simulink model "comparisonsPID"  (R2022b)
settings: Solver=ode45  StartTime=0.0  StopTime=80000  FixedStep=1e-6  RelTol=1e-10  AbsTol=1e-10
settings Model: Creator=svens  LastModifiedBy=saraa
settings SolverCC: ZeroCrossAlgorithm=Adaptive
settings DebuggingCC: IgnoredZcDiagnostic=none

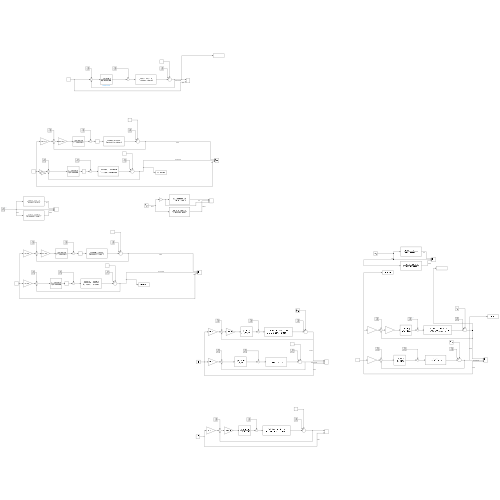
[thumbnail: Simulink's stored preview of the top-level diagram]
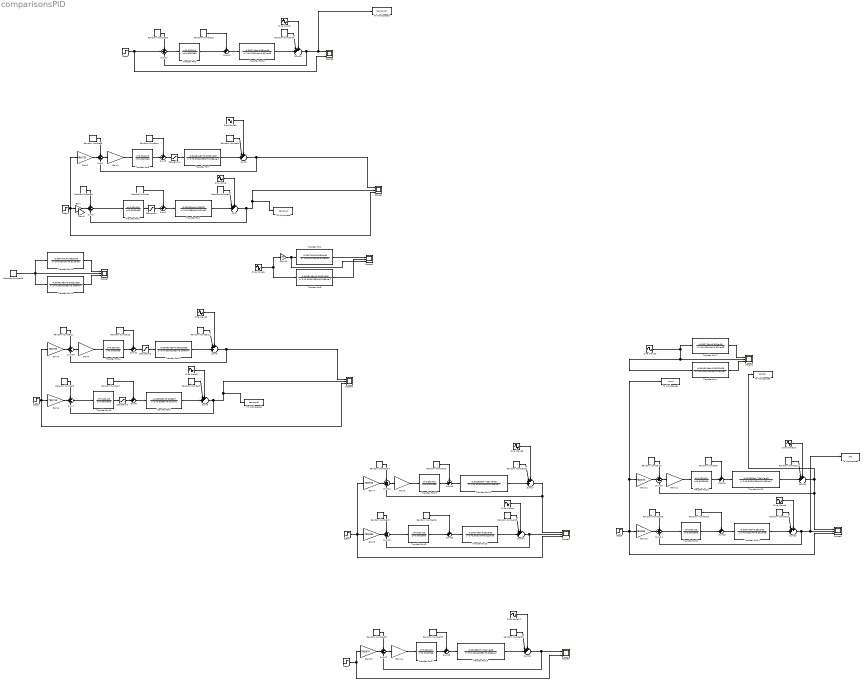
== system comparisonsPID ==
  Gain : Gain  Gain=1.05
  Gain{1,3..4,11,14} (5 alike) : Gain  Gain=0.0032072
  Gain10 : Gain  Gain=780
  Gain12 : Gain  Gain=780/675
  Gain13 : Gain  Gain=780/365
  Gain15 : Gain  Gain=780/675
  Gain2 : Gain  Gain=780/735
  Gain5 : Gain  Gain=780/735
  Gain6 : Gain  Gain=780/745
  Gain7 : Gain  Gain=780/675
  Gain8 : Gain  Gain=780/365
  Gain9 : Gain  Gain=1.05
  Random Number{,1,3..5,7..8,10..11,13..14,16..17,19..20,22..23,25..26,28..29} (21 alike) : RandomNumber  Variance=20  SampleTime=0.1
  Random Number{2,6,9,12,15,18,21,24,27,30} (10 alike) : RandomNumber  Variance=20  SampleTime=7800
  Saturation : Saturate  UpperLimit=100000  LowerLimit=50
  Saturation1 : Saturate  UpperLimit=2  LowerLimit=0  LinearizeAsGain=off
  Saturation2 : Saturate  UpperLimit=100000  LowerLimit=-10000
  Saturation3 : Saturate  UpperLimit=2  LowerLimit=0  LinearizeAsGain=off
  Scope{1..5,7..8} (7 alike) : Scope  NumInputPorts=3
  Scope6 : Scope  NumInputPorts=2
  Scope9 : Scope  NumInputPorts=2
  Sine Wave{,1..5,7..8,10,12} (10 alike) : Sin  Amplitude=6  Bias=25  Frequency=7.2e-5  SampleTime=0
  Sine Wave6 : Sin  SampleTime=0
  Sine Wave9 : Sin  SampleTime=0
  Step{1..6} (6 alike) : Step  After=780  SampleTime=0
  Sum{,3,6,9,14,17,20,23,26,32} (10 alike) : Sum  Inputs=+++||
  Sum{1,4,7,10,12,15,18,21,24,27} (10 alike) : Sum  Inputs=++-
  Sum{2,5,8,11,13,16,19,22,25,28} (10 alike) : Sum  Inputs=++|
  To Workspace : ToWorkspace  VariableName=tempout  SaveFormat=Timeseries  SampleTime=-1
  To Workspace1 : ToWorkspace  VariableName=tempout1  SaveFormat=Timeseries  SampleTime=-1
  To Workspace3 : ToWorkspace  VariableName=tempout3  SaveFormat=Timeseries  SampleTime=-1
  To Workspace4 : ToWorkspace  VariableName=input  SaveFormat=Timeseries  SampleTime=-1
  To Workspace5 : ToWorkspace  VariableName=red  SaveFormat=Timeseries  SampleTime=-1
  To Workspace6 : ToWorkspace  VariableName=control  SaveFormat=Timeseries  SampleTime=-1
  Transfer Fcn{1,16..18,20,24} (6 alike) : TransferFcn  Numerator=[-0.000749 9.681e-06]  Denominator=[1 0.02014 9.321e-05]
  Transfer Fcn{3,5,8,10,12..13,15,21,23,27} (10 alike) : TransferFcn  Numerator=[1 0.002419]  Denominator=[1 0.0002966]
  Transfer Fcn{4,6..7,11,19} (5 alike) : TransferFcn  Numerator=[-0.0648148 0.00021605]  Denominator=[1 0.00342593 3.0864e-7]
  Transfer Fcn14 : TransferFcn  Numerator=[-0.022685 7.5617e-05]  Denominator=[1 0.00342593 3.0864e-7]
  Transfer Fcn2 : TransferFcn  Numerator=[-0.009309 0.003657]  Denominator=[1 0.3965 0.001461]
  Transfer Fcn22 : TransferFcn  Numerator=[-0.022685 7.5617e-05]  Denominator=[1 0.00342593 3.0864e-7]
  Transfer Fcn26 : TransferFcn  Numerator=[-0.022685 7.5617e-05]  Denominator=[1 0.00342593 3.0864e-7]
  Transfer Fcn9 : TransferFcn  Numerator=[-0.009309 0.003657]  Denominator=[1 0.3965 0.001461]
  wires:
  Sum/1 -> Sum1/3, Scope1/2, To Workspace/1  "red neuronal"
  Transfer Fcn2/1 -> Sum/3
  Random Number/1 -> Sum2/1
  Random Number1/1 -> Sum1/1
  Sum2/1 -> Transfer Fcn2/1
  Sine Wave/1 -> Sum/1
  Random Number2/1 -> Sum/2
  Gain/1 -> Sum1/2
  Sum1/1 -> Transfer Fcn3/1
  Transfer Fcn3/1 -> Saturation/1
  Saturation/1 -> Sum2/2
  Transfer Fcn17/1 -> Scope2/1  "red"
  Transfer Fcn4/1 -> Scope2/3  "control"
  Sine Wave9/1 -> Transfer Fcn4/1, Scope2/2, Transfer Fcn17/1  "input"
  Transfer Fcn1/1 -> Scope3/1  "red"
  Sine Wave6/1 -> Gain10/1, Transfer Fcn6/1  "input"
  Transfer Fcn6/1 -> Scope3/2  "control"
  Step1/1 -> Gain2/1, Scope1/3, Gain/1  "input"
  Sine Wave1/1 -> Sum3/1
  Random Number6/1 -> Sum3/2
  Gain1/1 -> Transfer Fcn8/1
  Sum3/1 -> Scope1/1, Sum4/3  "control"
  Random Number4/1 -> Sum5/1
  Transfer Fcn8/1 -> Sum5/2
  Transfer Fcn7/1 -> Sum3/3
  Random Number5/1 -> Sum4/1
  Saturation1/1 -> Transfer Fcn7/1
  Sum4/1 -> Gain1/1
  Gain2/1 -> Sum4/2
  Sum5/1 -> Saturation1/1
  Sum9/1 -> Scope4/1, Sum10/3  "control"
  Gain4/1 -> Transfer Fcn12/1
  Random Number12/1 -> Sum9/2
  Sine Wave3/1 -> Sum9/1
  Sum11/1 -> Saturation3/1
  Saturation3/1 -> Transfer Fcn11/1
  Gain5/1 -> Sum10/2
  Transfer Fcn11/1 -> Sum9/3
  Transfer Fcn12/1 -> Sum11/2
  Random Number11/1 -> Sum10/1
  Random Number10/1 -> Sum11/1
  Transfer Fcn10/1 -> Saturation2/1
  Sine Wave2/1 -> Sum6/1
  Sum10/1 -> Gain4/1
  Sum6/1 -> Scope4/2, To Workspace1/1, Sum7/3  "red neuronal"
  Random Number9/1 -> Sum6/2
  Saturation2/1 -> Sum8/2
  Sum8/1 -> Transfer Fcn9/1
  Step2/1 -> Gain6/1, Gain5/1, Scope4/3  "input"
  Random Number7/1 -> Sum8/1
  Sum7/1 -> Transfer Fcn10/1
  Random Number8/1 -> Sum7/1
  Gain6/1 -> Sum7/2
  Transfer Fcn9/1 -> Sum6/3
  Gain10/1 -> Scope3/3, Transfer Fcn1/1
  Random Number24/1 -> Sum20/2
  Sum20/1 -> To Workspace3/1, Scope6/1, Sum21/3  "red neuronal"
  Sum21/1 -> Transfer Fcn5/1
  Transfer Fcn20/1 -> Sum20/3
  Random Number23/1 -> Sum21/1
  Step3/1 -> Sum21/2, Scope6/2  "input"
  Sine Wave7/1 -> Sum20/1
  Transfer Fcn5/1 -> Sum22/2
  Sum22/1 -> Transfer Fcn20/1
  Random Number22/1 -> Sum22/1
  Transfer Fcn18/1 -> Scope7/1  "red"
  Random Number19/1 -> Transfer Fcn19/1, Transfer Fcn18/1, Scope7/2  "input"
  Transfer Fcn19/1 -> Scope7/3  "control"
  Transfer Fcn21/1 -> Sum25/2
  Sum19/1 -> Transfer Fcn22/1
  Sum24/1 -> Transfer Fcn21/1
  Random Number27/1 -> Sum23/2
  Transfer Fcn23/1 -> Sum19/2
  Sum23/1 -> To Workspace5/1, Scope8/2, Sum24/3  "red neuronal"
  Random Number3/1 -> Sum19/1
  Sum26/1 -> Scope8/1, Sum18/3, To Workspace6/1  "control"
  Random Number21/1 -> Sum26/2
  Transfer Fcn24/1 -> Sum23/3
  Gain12/1 -> Sum18/2
  Sum18/1 -> Gain11/1
  Transfer Fcn22/1 -> Sum26/3
  Gain13/1 -> Sum24/2
  Random Number26/1 -> Sum24/1
  Gain11/1 -> Transfer Fcn23/1
  Step5/1 -> To Workspace4/1, Gain12/1, Scope8/3, Gain13/1  "input"
  Sine Wave10/1 -> Sum26/1
  Sine Wave8/1 -> Sum23/1
  Random Number20/1 -> Sum18/1
  Sum25/1 -> Transfer Fcn24/1
  Random Number25/1 -> Sum25/1
  Transfer Fcn13/1 -> Sum16/2
  Sum13/1 -> Transfer Fcn14/1
  Sum15/1 -> Transfer Fcn13/1
  Random Number18/1 -> Sum14/2
  Transfer Fcn15/1 -> Sum13/2
  Sum14/1 -> Scope5/2, Sum15/3  "red neuronal"
  Random Number13/1 -> Sum13/1
  Sum17/1 -> Scope5/1, Sum12/3  "control"
  Random Number15/1 -> Sum17/2
  Transfer Fcn16/1 -> Sum14/3
  Gain7/1 -> Sum12/2
  Sum12/1 -> Gain3/1
  Transfer Fcn14/1 -> Sum17/3
  Gain8/1 -> Sum15/2
  Random Number17/1 -> Sum15/1
  Gain3/1 -> Transfer Fcn15/1
  Step4/1 -> Gain7/1, Scope5/3, Gain8/1  "input"
  Sine Wave5/1 -> Sum17/1
  Sine Wave4/1 -> Sum14/1
  Random Number14/1 -> Sum12/1
  Sum16/1 -> Transfer Fcn16/1
  Random Number16/1 -> Sum16/1
  Transfer Fcn27/1 -> Sum28/2
  Random Number30/1 -> Sum32/2
  Gain15/1 -> Sum27/2
  Random Number28/1 -> Sum28/1
  Sum32/1 -> Sum27/3, Scope9/1
  Sum28/1 -> Transfer Fcn26/1
  Sine Wave12/1 -> Sum32/1
  Transfer Fcn26/1 -> Sum32/3
  Gain14/1 -> Transfer Fcn27/1
  Step6/1 -> Scope9/2, Gain15/1  "input"
  Sum27/1 -> Gain14/1
  Random Number29/1 -> Sum27/1
